simulink model "Standalone_CircuitSimulation"  (R2024b)
settings: Solver=FixedStepAuto  StartTime=0.0  StopTime=inf  RelTol=1e-3  EnableMultiTasking=on
undefined symbols (not defined in the file): IO397, pull, SensorCurrent_VoltAtZero, SensorCurrent_VoltPerAmp, up
libraries: nesl_utility x8, ee_lib x5, fl_lib x1, speedgoatlib_fpga_pwm x1, speedgoatlib_fpga x1, speedgoatlib_fpga_analog_io x1
settings Model: DataDictionary=SimulationData.sldd  Creator=rodri  LastModifiedBy=rodri
settings SolverCC: ConcurrentTasks=on  PositivePriorityOrder=on  AutoInsertRateTranBlk=on
settings OptimizationCC: BlockReduction=off  OptimizeBlockIOStorage=off
settings DebuggingCC: TasksWithSamePriorityMsg=none
settings HardwareCC: ProdBitPerLong=64  ProdLongLongMode=on  ProdHWDeviceType=Intel->x86-64 (Linux 64)
settings RTWCC: Description=Speedgoat Real-Time Target Machine  SystemTargetFile=speedgoat.tlc  TemplateMakefile=slrealtime_default_tmf  Toolchain=Simulink Real-Time Toolchain  BuildConfiguration=Faster Runs  CodeExecutionProfiling=on  TargetLang=C++
settings SimulinkRealTimeTargetCC: InstructionSetFMA=off  LogToMDFFile=off

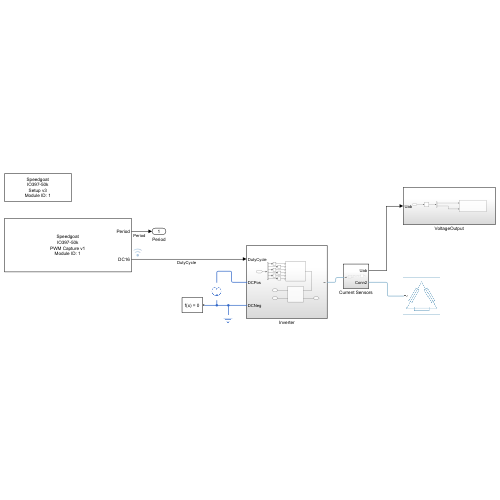
[thumbnail: Simulink's stored preview of the top-level diagram]
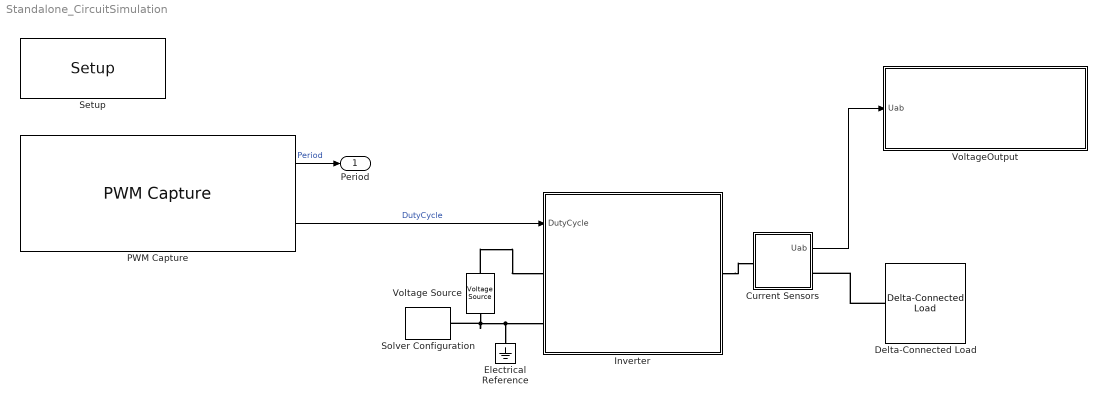
== system Standalone_CircuitSimulation ==
  Current Sensors : Subsystem
  Delta-Connected Load : ee_lib/Passive/RLC Assemblies/Delta-Connected Load  port_option=ee.enum.threePhasePort.composite  parameterization=ee.enum.rlc.parameterization.ratedpower  component_structure=ee.enum.rlc.structure.R  component_structure_PQ=ee.enum.rlc.structure.SeriesRL  R=1 Ohm  L=1e-3 H  C=1e-6 F  VRated=600 V  FRated=60 Hz  P=10e3 W  Qpos=1e3 A*V  Qneg=-1e2 A*V  R_parasitic=0 Ohm  G_parasitic=0 1/Ohm  R_parasitic_PQ=0 Ohm  G_parasitic_PQ=0 1/Ohm  Vmag0=24e3 V  Vang0=0 deg  Freq0=60 Hz  IL_specify=off  IL_priority=High  IL=[0, 0, 0] A  IL_nominal_specify=off  IL_nominal_value=1  IL_nominal_unit=A  VC_specify=off  VC_priority=High  VC=[0, 0, 0] V  VC_nominal_specify=off  VC_nominal_value=1  VC_nominal_unit=V
      settings: InternalSimscapePortConfiguration="{\"Bottom\":[],\"Left\":[{\"id\":\"N\",\"label\":\"~\",\"type\":\"foundation.electrical.three_phase\"}],\"Right\":[],\"Top\":[]}"
  Electrical Reference : fl_lib/Electrical/Electrical Elements/Electrical Reference
  Inverter : Subsystem
  PWM Capture : speedgoatlib_fpga_pwm/PWM Capture  id=1  chan=[2 6 4 1 5 3]  ts=0.0002  enableDma=on  captureMode=High transitions triggered  bit_width_cap=24  captureTimeout_si=0  captureTimeout_eff=[0]  debounce_si=1e-8  debounce_eff=[13.33e-9]  showHighDuration=off  showLowDuration=off  showPeriod=on  showDC16=on  showDC8=off  showTOn=off  showTOff=off  showValidData=off
      settings: SourceProductName=PWM
  Setup : speedgoatlib_fpga/Setup/Setup  Parameter124={}  board=IO397-50k  id=1  pciSlot=-1  device_id=1  bitstreamFilePath=C:\ProgramData\Speedgoat\bitstreams\io_configuration_package\R2024b\io397  bitstreamFile=speedgoat_IO397_HIL.mat  rearEnb_1=off  rearIO_1=None  rearEnb_2=off  rearIO_2=None  ProgSpiFlash=off  ProgBPIFlash=off  useFpgaDmaController=off  PullRPort15=pull-up 3.3V  PullRPort31=pull-up 3.3V  PullRPort47=pull-up 3.3V  PullRPort63=pull-up 3.3V  diffLineTermination_1=on  diffLineTermination_2=on  diffLineTermination_3=on  diffLineTermination_4=on  diffLineTermination_5=on  diffLineTermination_6=on  diffLineTermination_7=on  diffLineTermination_8=on  diffLineTermination_9=on  diffLineTermination_10=on  diffLineTermination_11=on  diffLineTermination_12=on  diffLineTermination_13=on  diffLineTermination_14=on  diffLineTermination_15=on  diffLineTermination_16=on  diffLineTermination_17=on  diffLineTermination_18=on  diffLineTermination_19=on  diffLineTermination_20=on  diffLineTermination_21=on  diffLineTermination_22=on  diffLineTermination_23=on  diffLineTermination_24=on  diffLineTermination_25=on  diffLineTermination_26=on  diffLineTermination_27=on  diffLineTermination_28=on  diffLineTermination_29=on  diffLineTermination_30=on  diffLineTermination_31=on  diffLineTermination_32=on  Vi_Pull_36x_1=Floating  Vo_36x_1=3.3V  Vi_Pull_36x_2=Floating  Vo_36x_2=3.3V  Vi_Pull_36x_3=Floating  Vo_36x_3=3.3V  Vi_Pull_36x_4=Floating  Vo_36x_4=3.3V  Vi_Pull_36x_5=Floating  Vo_36x_5=3.3V  Vi_Pull_36x_6=Floating  Vo_36x_6=3.3V  Vi_Pull_36x_7=Floating  Vo_36x_7=3.3V  Vi_Pull_36x_8=Floating  Vo_36x_8=3.3V  Vi_Pull_36x_9_16=Floating  Vo_36x_9_16=3.3V  Vi_Pull_36x_17_24=Floating  Vo_36x_17_24=3.3V  Vi_Pull_36x_25_32=Floating  Vo_36x_25_32=3.3V  Vi_Pull_36x_33_40=Floating  Vo_36x_33_40=3.3V  Vi_Pull_36x_41_48=Floating  Vo_36x_41_48=3.3V  Vi_Pull_36x_49_56=Floating  Vo_36x_49_56=3.3V  Vi_Pull_36x_57_64=Floating  Vo_36x_57_64=3.3V  PullRPort0_1=pull-up  VioPort0_1=3.3V  PullRPort1_1=pull-up  VioPort1_1=3.3V  PullRPort2_1=pull-up  VioPort2_1=3.3V  PullRPort3_1=pull-up  VioPort3_1=3.3V  PullRPort4_1=pull-up  VioPort4_1=3.3V  PullRPort5_1=pull-up  VioPort5_1=3.3V  PullRPort6_1=pull-up  VioPort6_1=3.3V  diffLineTermination_rear1_1=on  diffLineTermination_rear1_2=on  diffLineTermination_rear1_3=on  diffLineTermination_rear1_4=on  diffLineTermination_rear1_5=on  diffLineTermination_rear1_6=on  diffLineTermination_rear1_7=on  diffLineTermination_rear1_8=on  PullRPort0_2=pull-up  VioPort0_2=3.3V  PullRPort1_2=pull-up  VioPort1_2=3.3V  PullRPort2_2=pull-up  VioPort2_2=3.3V  PullRPort3_2=pull-up  VioPort3_2=3.3V  PullRPort4_2=pull-up  VioPort4_2=3.3V  PullRPort5_2=pull-up  VioPort5_2=3.3V  PullRPort6_2=pull-up  VioPort6_2=3.3V  diffLineTermination_rear2_1=on  diffLineTermination_rear2_2=on  diffLineTermination_rear2_3=on  diffLineTermination_rear2_4=on  diffLineTermination_rear2_5=on  diffLineTermination_rear2_6=on  diffLineTermination_rear2_7=on  diffLineTermination_rear2_8=on
      settings: SourceProductName=IO3xx
  Solver Configuration : nesl_utility/Solver Configuration  PhysicalDomain=network_engine_domain  SubClassName=solver  LeftPortType=input  RightPortType=generic  Tones=[]  Harmonics=[]  SimulateNoise=off  Profile=off  UseLocalSampling=off  EnableSwitchedLinearOptims=on  FrequencyDomain=off  UseCCode=off  RelTol=0.001  AbsTol=0.001  MinStep=1e-09  ToWorkspace=off  RevertToSquareIcSolve=off  NumHomotopyIterations=100  PhasorMode=off  PhasorModeNumHarmonics=1  ConsistencySolver=NEWTON_XTOL_AFTER_FTOL  IndexReductionMethod=DerivativeReplacement  DoDC=on  ResidualTolerance=1e-09  ConsistencyTolSource=GLOBAL  ConsistencyAbsTol=0.001  ConsistencyRelTol=0.001  ConsistencyTolFactor=0.005  UseLocalSolver=on  LocalSolverChoice=NE_PARTITIONING_ADVANCER  ResolveIndetEquations=on  FunctionEvalNumThread=1  LocalSolverSampleTime=0.0002  DoFixedCost=on  MaxNonlinIter=3  MaxModeIter=2  ComputeImpulses=off  ImpulseIterations=2  LinearAlgebra=auto  LinearAlgebraNumThread=0  EquationFormulation=NE_TIME_EF  DelaysMemoryBudget=1024  AutomaticFiltering=on  FilteringTimeConstant=0.001  PartitionStorageMethod=AS_NEEDED  PartitionMemoryBudget=1024  PartitionMethod=FAST  MultibodyUseLocalSolver=off  MultibodyLocalSolverChoice=ODE1  MultibodyLocalSolverSampleTime=0.001
  Voltage Source : ee_lib/Sources/Voltage Source  dc_voltage=DCV V  ac_voltage=0 V  ac_shift=0 rad  ac_frequency=60 Hz  noise_mode=ee.enum.sources.noise.Disabled  PSD=0 V^2/Hz  sample_time=1e-3 s  repeatability=ee.enum.sources.repeatability.NotRepeatable  user_seed=0  auto_seed=1632071392  i_specify=off  i_priority=None  i=0 A  i_nominal_specify=off  i_nominal_value=1  i_nominal_unit=A  v_specify=off  v_priority=None  v=0 V  v_nominal_specify=off  v_nominal_value=1  v_nominal_unit=V
  VoltageOutput : Subsystem
  Period : Outport
  wires:
  PWM Capture/1 -> Period/1  "Period"
  PWM Capture/2 -> Inverter/1(DutyCycle)  "DutyCycle"
  Current Sensors/1(Uab) -> VoltageOutput/1(Uab)
  connections:
  Voltage Source/RConn1 -- Solver Configuration/RConn1 -- Inverter/LConn2 -- Electrical Reference/LConn1
  Voltage Source/LConn1 -- Inverter/LConn1
  Inverter/RConn1 -- Current Sensors/LConn1
  Delta-Connected Load/LConn1 -- Current Sensors/RConn1

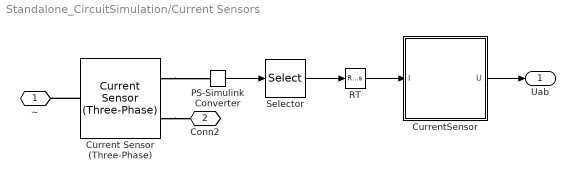
== system Standalone_CircuitSimulation/Current Sensors ==
  Current Sensor (Three-Phase) : ee_lib/Sensors & Transducers/Current Sensor (Three-Phase)
  CurrentSensor : Subsystem  TreatAsAtomicUnit=on  ScheduleAs=Periodic partition  PartitionName=CurrentSensor  SystemSampleTime=0.0002
  PS-Simulink Converter : nesl_utility/PS-Simulink Converter  PhysicalDomain=network_engine_domain  SubClassName=ps_output  LeftPortType=input  RightPortType=output  PseudoPeriodic=off  Frequencies=[]  VectorFormat=inherit  Unit=inherit  AffineConversion=off
  RT : RateTransition
  Selector : Selector  InputPortWidth=3  IndexOptions=Index vector (dialog)  Indices=[1 2]  OutputSizes=1
  ~ : PMIOPort  Side=Left
  Conn2 : PMIOPort  Port=2  Side=Right
  Uab : Outport
  wires:
  CurrentSensor/1(U) -> Uab/1
  PS-Simulink Converter/1 -> Selector/1
  Selector/1 -> RT/1
  RT/1 -> CurrentSensor/1(I)
  connections:
  Current Sensor (Three-Phase)/RConn1 -- PS-Simulink Converter/LConn1
  Current Sensor (Three-Phase)/LConn1 -- ~/RConn1
  Current Sensor (Three-Phase)/RConn2 -- Conn2/RConn1

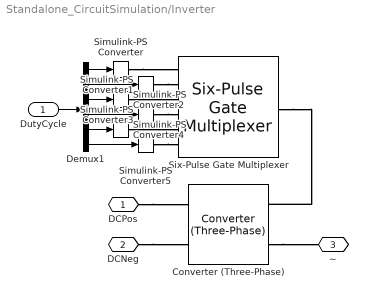
== system Standalone_CircuitSimulation/Inverter ==
  DutyCycle : Inport
  Converter (Three-Phase) : ee_lib/Semiconductors & Converters/Converters/Converter (Three-Phase)  port_option=ee.enum.threePhasePort.composite  fidelity_option=ee.enum.converters.fidelity.detailed  device_type=ee.enum.converters.switchingdevice.averaged  showThermalPort=false  K=0  Vth=6 V  Vgt=1 V  Vgt_off=-1 V  Ih=1 A  Vf=0.8 V  Ron=0.001 Ohm  Rds=0.001 Ohm  Goff=1e-6 1/Ohm  Eon_scalar=22.86e-3 J  Eoff_scalar=17.14e-3 J  Eoff_natural_commutation=10e-3 J  Voff=300 V  Iout_scalar=600 A  onCurrentMeasDelay=0 s  useCurrentFromPreviousCycle=false  useVoltageFromPreviousCycle=false  diode_param=ee.enum.converters.protectiondiode.none  diode_Vf=0.8 V  diode_Ron=0.001 Ohm  diode_Goff=1e-5 1/Ohm  diode_C=50 nF  diode_iRM=-235 A  diode_iF=300 A  diode_idot=-50 A/us  diode_trr_param=ee.enum.converters.diodetrr.trr_factor  diode_trr_factor=3  diode_trr=15 us  diode_Qrr=1500 s*uA  diode_rec_loss_model=ee.enum.diode.reverseRecoveryModel.fixed  diode_ErecVal=0 J  diode_scaleWithIandV=false  diode_ErecMat=zeros(2, 3) J  diode_TjrecVec=[298.15, 398.15] K  diode_IfrecVec=[.1, 1, 10] A  diode_IrecVal=10 A  diode_VrecVal=10 V  diode_tFilter=1 / 1000 / 100 s  thermal_network_parameterization=ee.enum.thermalNetworkTopology.external  Rth=[.08, .5] K/W  Rth_Cauer=[.08, .1, .5] K/W  Rth_Foster=[.08, .14, .22, .16] K/W  thermal_mass_parameterization=ee.enum.thermalNetwork.timeconstant  thermal_mass=[.01, .5] J/K  thermal_mass_Cauer=[.01, .1, .5] J/K  thermal_mass_Foster=[.001, .005, .05, .5] J/K  thermal_time_constant=[.001, .2] s  thermal_time_constant_Cauer=[.001, .1, .2] s  thermal_time_constant_Foster=[7e-05, .0007, .01, .08] s  thermal_mass_initial_temperatures=[25, 25] degC  thermal_mass_initial_temperatures_Cauer=[25, 25, 25] degC  junction_thermal_mass=0.01 J/K  Tvec_initial_Foster=[25, 25, 25, 25] degC  snubber_type=ee.enum.converters.snubber.exclude  Cs=1e-7 F  Rs=0.1 Ohm  Vce_loss=[0, 150, 300] V
  Demux1 : Demux  Outputs=6
  Simulink-PS Converter{,1..5} (6 alike) : nesl_utility/Simulink-PS Converter  PhysicalDomain=network_engine_domain  SubClassName=ps_input  LeftPortType=input  RightPortType=output  PseudoPeriodic=off  Frequencies=[]  NoiseDistribution=none  NoiseParameters=[]  Unit=1  AffineConversion=off  FilteringAndDerivatives=provide  SimscapeFilterOrder=1  InputFilterTimeConstant=0.001  UdotUserProvided=0
  Six-Pulse Gate Multiplexer : ee_lib/Semiconductors & Converters/Converters/Six-Pulse Gate Multiplexer  port_option=ee.enum.controlport.ps
  DCPos : PMIOPort  Side=Left
  DCNeg : PMIOPort  Port=2  Side=Left
  ~ : PMIOPort  Port=3  Side=Right
  wires:
  Demux1/2 -> Simulink-PS Converter1/1
  Demux1/4 -> Simulink-PS Converter3/1
  Demux1/1 -> Simulink-PS Converter/1
  Demux1/3 -> Simulink-PS Converter2/1
  DutyCycle/1 -> Demux1/1
  Demux1/6 -> Simulink-PS Converter5/1
  Demux1/5 -> Simulink-PS Converter4/1
  connections:
  Simulink-PS Converter1/RConn1 -- Six-Pulse Gate Multiplexer/LConn2
  Simulink-PS Converter3/RConn1 -- Six-Pulse Gate Multiplexer/LConn4
  Simulink-PS Converter5/RConn1 -- Six-Pulse Gate Multiplexer/LConn6
  DCPos/RConn1 -- Converter (Three-Phase)/RConn1
  Simulink-PS Converter/RConn1 -- Six-Pulse Gate Multiplexer/LConn1
  Simulink-PS Converter2/RConn1 -- Six-Pulse Gate Multiplexer/LConn3
  Simulink-PS Converter4/RConn1 -- Six-Pulse Gate Multiplexer/LConn5
  DCNeg/RConn1 -- Converter (Three-Phase)/RConn2
  Six-Pulse Gate Multiplexer/RConn1 -- Converter (Three-Phase)/LConn1
  Converter (Three-Phase)/LConn2 -- ~/RConn1

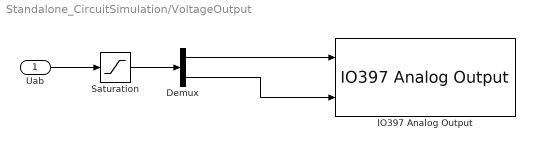
== system Standalone_CircuitSimulation/VoltageOutput ==
  Uab : Inport
  Demux : Demux  Outputs=2
  IO397 Analog Output : speedgoatlib_fpga_analog_io/IO397/IO397 Analog Output  id=1  chan=[1 2]  initVal=0  resetVal=0  ts=0.0002  span=+5 V
      settings: SourceProductName=Analog IO
  Saturation : Saturate  UpperLimit=3.3  LowerLimit=0
  wires:
  Demux/2 -> IO397 Analog Output/2
  Demux/1 -> IO397 Analog Output/1
  Uab/1 -> Saturation/1
  Saturation/1 -> Demux/1

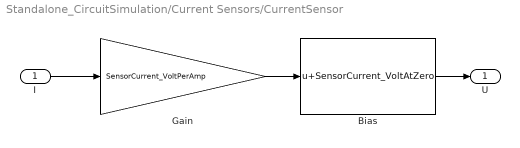
== system Standalone_CircuitSimulation/Current Sensors/CurrentSensor ==
  I : Inport
  Bias : Bias  Bias=SensorCurrent_VoltAtZero  SaturateOnIntegerOverflow=off
  Gain : Gain  Gain=SensorCurrent_VoltPerAmp
  U : Outport
  wires:
  I/1 -> Gain/1
  Gain/1 -> Bias/1
  Bias/1 -> U/1
